simulink model "convertidorsimu"  (R2026a)
settings: Solver=VariableStepAuto  StopTime=0.005
settings Model: Creator=ghass  LastModifiedBy=ghass

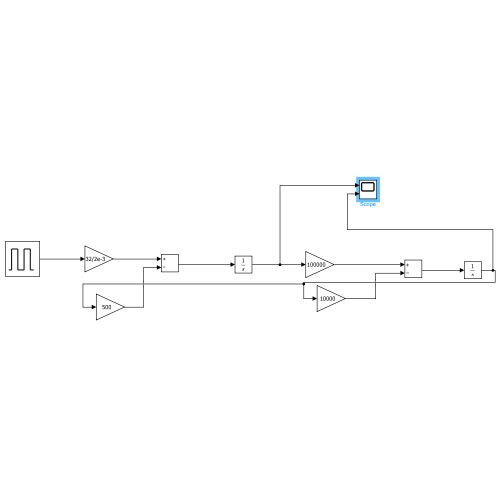
[thumbnail: Simulink's stored preview of the top-level diagram]
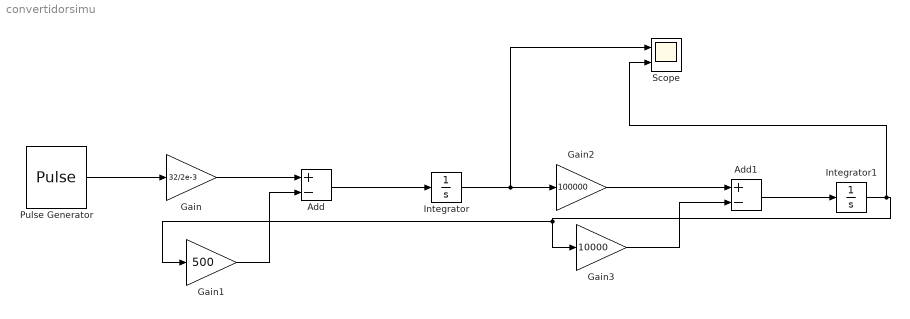
== system convertidorsimu ==
  Add : Sum  Inputs=+-
  Add1 : Sum  Inputs=+-
  Gain : Gain  Gain=32/2e-3
  Gain1 : Gain  Gain=500
  Gain2 : Gain  Gain=100000
  Gain3 : Gain  Gain=10000
  Integrator : Integrator
  Integrator1 : Integrator
  Pulse Generator : DiscretePulseGenerator  PulseType=Time based  Period=1/100e3  PulseWidth=40
  Scope : Scope  NumInputPorts=2
      settings: ActiveDisplayYMinimum=-0.22923056525229946  ActiveDisplayYMaximum=14.27198036058134
  wires:
  Pulse Generator/1 -> Gain/1
  Gain/1 -> Add/1
  Add/1 -> Integrator/1
  Integrator/1 -> Scope/1, Gain2/1
  Gain2/1 -> Add1/1
  Gain1/1 -> Add/2
  Gain3/1 -> Add1/2
  Add1/1 -> Integrator1/1
  Integrator1/1 -> Scope/2, Gain1/1, Gain3/1
